simulink model "case_02_slow_steady"  (R2025b)
settings: Solver=VariableStepAuto  StartTime=0.0  StopTime=60  RelTol=1e-3
settings Model: Creator=sanborkl  LastModifiedBy=sanborkl

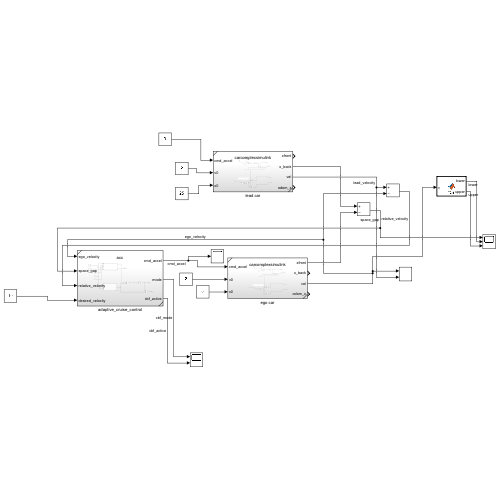
[thumbnail: Simulink's stored preview of the top-level diagram]
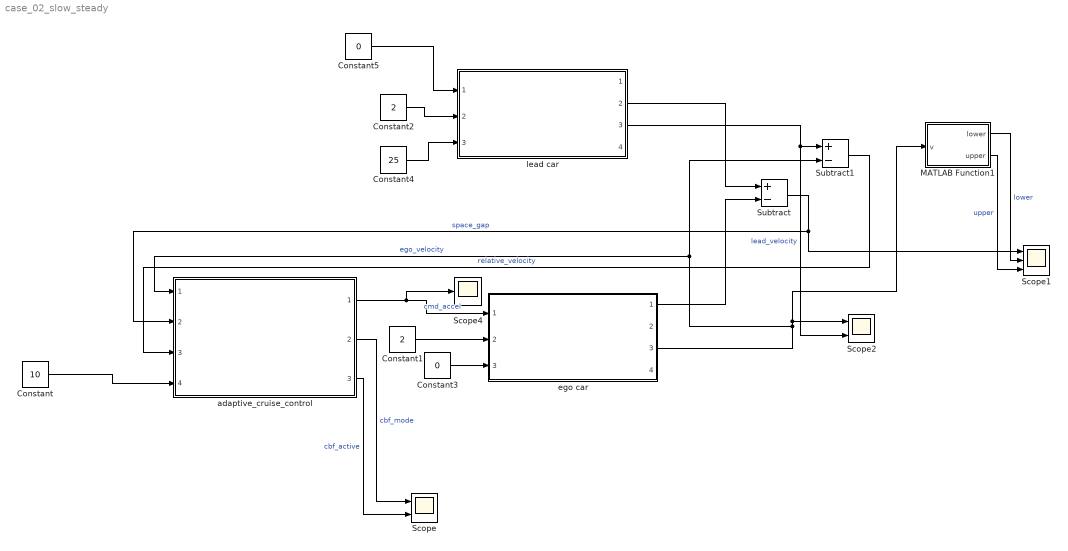
== system case_02_slow_steady ==
  Constant : Constant  Value=10
  Constant1 : Constant  Value=2
  Constant2 : Constant  Value=2
  Constant3 : Constant  Value=0
  Constant4 : Constant  Value=25
  Constant5 : Constant  Value=0
  MATLAB Function1 : MATLAB Function  TreatAsAtomicUnit=on
  Scope : Scope  NumInputPorts=2
      settings: ActiveDisplayYMinimum=0.875  ActiveDisplayYMaximum=2.125
  Scope1 : Scope  NumInputPorts=3
      settings: ActiveDisplayYMinimum=6.9050000000000011  ActiveDisplayYMaximum=27.854999999999997  YLabel=m
  Scope2 : Scope  NumInputPorts=2
      settings: ActiveDisplayYMinimum=1.6532107581563631  ActiveDisplayYMaximum=2.842411479479614  YLabel=m/s  DataLoggingVariableName=ScopeData2
  Scope4 : Scope
      settings: ActiveDisplayYMinimum=-0.24475000000000013  ActiveDisplayYMaximum=0.58275  YLabel=m/s^2  DataLoggingVariableName=ScopeData6
  Subtract : Sum  Inputs=+-
  Subtract1 : Sum  Inputs=+-
  adaptive_cruise_control : Subsystem  ReferencedSubsystem=acc
  ego car : Subsystem  ReferencedSubsystem=carcomplexsimulink
  lead car : Subsystem  ReferencedSubsystem=carcomplexsimulink
  wires:
  MATLAB Function1/1(lower) -> Scope1/2  "lower"
  lead car/2 -> Subtract/1
  adaptive_cruise_control/2 -> Scope/1  "cbf_mode"
  MATLAB Function1/2(upper) -> Scope1/3  "upper"
  adaptive_cruise_control/3 -> Scope/2  "cbf_active"
  Constant/1 -> adaptive_cruise_control/4
  Subtract1/1 -> adaptive_cruise_control/3  "relative_velocity"
  Constant2/1 -> lead car/2
  lead car/3 -> Scope2/2, Subtract1/1  "lead_velocity"
  Constant3/1 -> ego car/3
  Constant4/1 -> lead car/3
  Subtract/1 -> Scope1/1, adaptive_cruise_control/2  "space_gap"
  ego car/1 -> Subtract/2
  adaptive_cruise_control/1 -> Scope4/1, ego car/1  "cmd_accel"
  Constant5/1 -> lead car/1
  ego car/3 -> Scope2/1, MATLAB Function1/1(v), adaptive_cruise_control/1, Subtract1/2  "ego_velocity"
  Constant1/1 -> ego car/2

== matlab function case_02_slow_steady/MATLAB Function1 ==
  data: v input; lower output; upper output
function [lower, upper] = fcn(v)

lower = 2 * v + 5;
upper = 2 * v + 15;
